simulink model "DRLHevIps"  (R2025b)
settings: Solver=ode23tb  StartTime=0  StopTime=stop_time+1  FixedStep=ts  RelTol=1e-3  AbsTol=1e-4
model workspace (MAT data in the model file):
  BattChrgMax = Simulink.Parameter
  BattChrgMax.Value = -28000
  BattChrgMax.Complexity = 'real'
  BattChrgMax.Dimensions = [1 1]
  BattChrgMax.DataType = 'double'
  BattDischrgMax = Simulink.Parameter
  BattDischrgMax.Value = 28000
  BattDischrgMax.Complexity = 'real'
  BattDischrgMax.Dimensions = [1 1]
  BattDischrgMax.DataType = 'double'
  BrkPrsMax = Simulink.Parameter
  BrkPrsMax.Value = 5000000
  BrkPrsMax.Complexity = 'real'
  BrkPrsMax.Dimensions = [1 1]
  BrkPrsMax.DataType = 'double'
  DiffRatio = Simulink.Parameter
  DiffRatio.Value = 3.267
  DiffRatio.Complexity = 'real'
  DiffRatio.Dimensions = [1 1]
  DiffRatio.DataType = 'double'
  EVSpdLmt = Simulink.Parameter
  EVSpdLmt.Value = 16
  EVSpdLmt.Complexity = 'real'
  EVSpdLmt.Dimensions = [1 1]
  EVSpdLmt.DataType = 'double'
  EngIdle = Simulink.Parameter
  EngIdle.Value = 78.5398163397
  EngIdle.Complexity = 'real'
  EngIdle.Dimensions = [1 1]
  EngIdle.DataType = 'double'
  EngPwr = Simulink.Parameter
  EngPwr.Value = [8377.58040957 15052.6315789 19736.8421053 24421.0526316 29105.2631579 33789.4736842 38473.6842105 43157.8947368 47842.1052632 52526.3157895 57210.5263158 61894.7368421 66578.9473684 71263.1578947 75947.3684211 80631.5789474 85315.7894737 90000]
  EngPwr.Complexity = 'real'
  EngPwr.Dimensions = [1 18]
  EngPwr.DataType = 'double'
  EngSpd = Simulink.Parameter
  EngSpd.Value = [1000 1448.84862461 1712.99052669 1980.33600187 2249.1155588 2517.55970613 2783.89895252 3046.3638066 3303.18477703 3552.59237246 3792.81710154 4022.08947291 4238.63999523 4440.69917715 4626.49752731 4794.26555436 4942.23376695 5068.63267374]
  EngSpd.Complexity = 'real'
  EngSpd.Dimensions = [1 18]
  EngSpd.DataType = 'double'
  EngTrq = Simulink.Parameter
  EngTrq.Value = [80 99.2112225513 110.02568665 117.759751017 123.57514891 128.166058939 131.971967205 135.285068696 138.308475993 141.18967656 144.040766791 146.951280713 149.9967243 153.244568751 156.75874496 160.603298419 164.845657961 169.559869104]
  EngTrq.Complexity = 'real'
  EngTrq.Dimensions = [1 18]
  EngTrq.DataType = 'double'
  EngTrqWhl = Simulink.Parameter
  EngTrqWhl.Value = [87.7908306305 126.105850222 164.420869813 193.843356507 202.735889404 240.750809081 272.197383842 292.721746259 307.117840187 318.924150962 329.429038197 339.950469104 351.800120347 366.619114839 388.284464425 404.750071694]
  EngTrqWhl.Complexity = 'real'
  EngTrqWhl.Dimensions = [1 16]
  EngTrqWhl.DataType = 'double'
  GenMapEff = Simulink.Parameter
  GenMapEff.Value = [60  60  60  60  60  65  60  60  60  60  60  60  60  60  60; 60  78  85  87  88  89  91  91  93  92  92  93  91  90  85; 60  82  88  90  90.5  92.5  94.5  95  95  94.5  93.5  93  93  93  93; 60  82  89  91  91.5  93.5  95  95  94.5  94  93  93  93  93  93; 60  82  88  91  92  94  95  94  94  93  93  93  93  93  93; 60  80  88  90.5  91.5  94  94.5  94  93  93  93  93  93  93  93; 60  78  87  90  90.5  93  94  93  93  93  93  93  93  93  93; 60  75  86  89  90  92  92  92  92  92  92  92  92  92  92; 60  74  84  87.5  89  91  91  91  91  91  91  91  91  91  91; 60  70  81  86  88  88  88  88  88  88  88  88  88  88  88; 60  66  79  86  88  88  88  88  88  88  88  88  88  88  88; 60  66  79  86  88  88  88  88  88  88  88  88  88  88  88]
  GenMapEff.Complexity = 'real'
  GenMapEff.Dimensions = [12 15]
  GenMapEff.DataType = 'double'
  GenMapSpdIndex = Simulink.Parameter
  GenMapSpdIndex.Value = [0 1000 2000 2767.91 3000 4000 5000 6000 7000 8000 9000 10000 11000 12000 13000]
  GenMapSpdIndex.Complexity = 'real'
  GenMapSpdIndex.Dimensions = [1 15]
  GenMapSpdIndex.DataType = 'double'
  GenMapTrqIndex = Simulink.Parameter
  GenMapTrqIndex.Value = [0 14 28 42 56 70 84 98 112 126 140 144.9]
  GenMapTrqIndex.Complexity = 'real'
  GenMapTrqIndex.Dimensions = [1 12]
  GenMapTrqIndex.DataType = 'double'
  GenPwrMax = Simulink.Parameter
  GenPwrMax.Value = 42000
  GenPwrMax.Complexity = 'real'
  GenPwrMax.Dimensions = [1 1]
  GenPwrMax.DataType = 'double'
  GenSpd = Simulink.Parameter
  GenSpd.Value = [0 1000 2000 2767.91 3000 4000 5000 6000 7000 8000 9000 10000 11000 12000 13000 13500]
  GenSpd.Complexity = 'real'
  GenSpd.Dimensions = [1 16]
  GenSpd.DataType = 'double'
  GenTrq = Simulink.Parameter
  GenTrq.Value = [144.9 144.9 144.9 144.9 133.69015219 100.26761416 80.2140913 66.845076102 57.295779513 50.133807073 44.563384068 40.107045657 36.460950596 33.422538051 30.851573585 29.708922712]
  GenTrq.Complexity = 'real'
  GenTrq.Dimensions = [1 16]
  GenTrq.DataType = 'double'
  GenTrqMax = Simulink.Parameter
  GenTrqMax.Value = 144.9
  GenTrqMax.Complexity = 'real'
  GenTrqMax.Dimensions = [1 1]
  GenTrqMax.DataType = 'double'
  MotMapEff = Simulink.Parameter
  MotMapEff.Value = [60  60  60  60  60  65  60  60  60  60  60  60  60  60  60; 60  78  85  87  88  89  91  91  93  92  92  93  91  90  85; 60  82  88  90  90.5  92.5  94.5  95  95  94.5  93.5  93  93  93  93; 60  82  89  91  91.5  93.5  95  95  94.5  94  93  93  93  93  93; 60  82  88  91  92  94  95  94  94  93  93  93  93  93  93; 60  80  88  90.5  91.5  94  94.5  94  93  93  93  93  93  93  93; 60  78  87  90  90.5  93  94  93  93  93  93  93  93  93  93; 60  75  86  89  90  92  92  92  92  92  92  92  92  92  92; 60  74  84  87.5  89  91  91  91  91  91  91  91  91  91  91; 60  70  81  86  88  88  88  88  88  88  88  88  88  88  88; 60  66  79  86  88  88  88  88  88  88  88  88  88  88  88; 60  66  79  86  88  88  88  88  88  88  88  88  88  88  88]
  MotMapEff.Complexity = 'real'
  MotMapEff.Dimensions = [12 15]
  MotMapEff.DataType = 'double'
  MotMapSpdIndex = Simulink.Parameter
  MotMapSpdIndex.Value = [0 1000 2000 2767.91 3000 4000 5000 6000 7000 8000 9000 10000 11000 12000 13000]
  MotMapSpdIndex.Complexity = 'real'
  MotMapSpdIndex.Dimensions = [1 15]
  MotMapSpdIndex.DataType = 'double'
  MotMapTrqIndex = Simulink.Parameter
  MotMapTrqIndex.Value = [0 20 40 60 80 100 120 140 160 180 200 207]
  MotMapTrqIndex.Complexity = 'real'
  MotMapTrqIndex.Dimensions = [1 12]
  MotMapTrqIndex.DataType = 'double'
  MotPwr = Simulink.Parameter
  MotPwr.Value = [0 21676.9893098 43353.9786195 59999.9554804 59999.9999968 60000.0000072 59999.9999863 60000.0000031 59999.9999999 59999.9999989 60000.0000031 59999.9999968 59999.9999947 60000.0000031 60000.000002 60000.0000031]
  MotPwr.Complexity = 'real'
  MotPwr.Dimensions = [1 16]
  MotPwr.DataType = 'double'
  MotSpd = Simulink.Parameter
  MotSpd.Value = [0 1000 2000 2767.91 3000 4000 5000 6000 7000 8000 9000 10000 11000 12000 13000 13500]
  MotSpd.Complexity = 'real'
  MotSpd.Dimensions = [1 16]
  MotSpd.DataType = 'double'
  MotTrq = Simulink.Parameter
  MotTrq.Value = [207 207 207 207 190.9859317 143.2394488 114.591559 95.49296586 81.85111359 71.61972439 63.66197724 57.29577951 52.08707228 47.74648293 44.07367655 42.44131816]
  MotTrq.Complexity = 'real'
  MotTrq.Dimensions = [1 16]
  MotTrq.DataType = 'double'
  Ndiff = Simulink.Parameter
  Ndiff.Value = 3.26774691358
  Ndiff.Complexity = 'real'
  Ndiff.Dimensions = [1 1]
  Ndiff.DataType = 'double'
  Nr1 = Simulink.Parameter
  Nr1.Value = 78
  Nr1.Complexity = 'real'
  Nr1.Dimensions = [1 1]
  Nr1.DataType = 'double'
  Nr2 = Simulink.Parameter
  Nr2.Value = 58
  Nr2.Complexity = 'real'
  Nr2.Dimensions = [1 1]
  Nr2.DataType = 'double'
  Ns1 = Simulink.Parameter
  Ns1.Value = 30
  Ns1.Complexity = 'real'
  Ns1.Dimensions = [1 1]
  Ns1.DataType = 'double'
  Ns2 = Simulink.Parameter
  Ns2.Value = 22
  Ns2.Complexity = 'real'
  Ns2.Dimensions = [1 1]
  Ns2.DataType = 'double'
  NsysWhl = Simulink.Parameter
  NsysWhl.Value = [0 116.077026422 232.154052844 321.290762203 348.231079266 464.308105687 580.385132109 696.462158531 812.539184953 928.616211375 1044.6932378 1160.77026422 1276.84729064 1392.92431706 1509.00134348 1567.0398567]
  NsysWhl.Complexity = 'real'
  NsysWhl.Dimensions = [1 16]
  NsysWhl.DataType = 'double'
  SOCChrgFactor = Simulink.Parameter
  SOCChrgFactor.Value = [84000 8400]
  SOCChrgFactor.Complexity = 'real'
  SOCChrgFactor.Dimensions = [1 2]
  SOCChrgFactor.DataType = 'double'
  SOCerr = Simulink.Parameter
  SOCerr.Value = 20
  SOCerr.Complexity = 'real'
  SOCerr.Dimensions = [1 1]
  SOCerr.DataType = 'double'
  SOCmax = Simulink.Parameter
  SOCmax.Value = 80
  SOCmax.Complexity = 'real'
  SOCmax.Dimensions = [1 1]
  SOCmax.DataType = 'double'
  SOCmin = Simulink.Parameter
  SOCmin.Value = 40
  SOCmin.Complexity = 'real'
  SOCmin.Dimensions = [1 1]
  SOCmin.DataType = 'double'
  SOCtarget = Simulink.Parameter
  SOCtarget.Value = 60
  SOCtarget.Complexity = 'real'
  SOCtarget.Dimensions = [1 1]
  SOCtarget.DataType = 'double'
  SysTrqWhl = Simulink.Parameter
  SysTrqWhl.Value = [1783.29861111 1783.29861111 1783.29861111 1783.29861111 1783.29861111 1474.75423952 1259.40012785 1115.39069983 1012.2626575 935.925866097 877.875007244 833.551841194 800.528640413 777.953591624 767.977827605 770.380717725]
  SysTrqWhl.Complexity = 'real'
  SysTrqWhl.Dimensions = [1 16]
  SysTrqWhl.DataType = 'double'
  k = Simulink.Parameter
  k.Value = 2.6
  k.Complexity = 'real'
  k.Dimensions = [1 1]
  k.DataType = 'double'
values from neighbouring files (symbols this model uses):
  cyc_time = WLTC(:,1)    [mdlrun_time_DG.m]
  cyc_vel = WLTC(:,2)    [mdlrun_time_DG.m]
  en_actsmo = 1    [mdlrun_time_DG.m]
  en_elec = 1    [mdlrun_time_DG.m]
  en_gas = 1    [mdlrun_time_DG.m]
  en_SOCpen = 1    [mdlrun_time_DG.m]
  k_actsmo = 5e-2    (= 0.05)    [mdlrun_time_DG.m]
  k_elec = 1    [mdlrun_time_DG.m]
  k_gas = 1    [mdlrun_time_DG.m]
  k_SOCpen = 1.2    [mdlrun_time_DG.m]
  obs_max = 1e4*[0.0020, 0.0090, 0.0100, 0.0100, 8.4000, 0.0100,                0.0056, 0.1011, 2.8000,      0, 0.0001, 0.0132,                0.0740, 2.6065, 0.0339, 0.0949, 0.0117, 2.4444]    [mdlrun_time_DG.m]
  obs_min = 1e4*[0.0010, 0.0070,      0,      0, 0.8400,      0,                     0, -0.0005,     0, -2.8000,     0, -0.0032               -0.0694, -2.7092, -0.0030,    0, -0.0001, -2.7647]    [mdlrun_time_DG.m]
  Price_elec = 1    [mdlrun_time_DG.m]
  Price_gas = 7.14    [mdlrun_time_DG.m]
  rho_gas = 0.739    [mdlrun_time_DG.m]
  stop_time = cyc_time(end)    [mdlrun_time_DG.m]
  ts = 1    [mdlrun_time_DG.m]
undefined symbols (not defined in the file or in its folder): n_ool, T_ool
libraries: simulink x29, autolibutils x6, slpidlib x2, rllib x2, SignalEditorBlockLib x1, autolibshared x1, autolibhevctrlrcommon x1
(part 1 of 4)
settings Model: DataDictionary=HevIps.sldd  ModifiedByFormat=The MathWorks, Inc.  PauseTimes=23.46  Creator=The MathWorks, Inc.  LastModifiedBy=The MathWorks, Inc.
settings SolverCC: ExtrapolationOrder=1.0  NumberNewtonIterations=20.0  SolverJacobianMethodControl=FullPerturbation  ZeroCrossControl=EnableAll  ZeroCrossAlgorithm=Adaptive  AlgebraicLoopSolver=TrustRegion  AutoInsertRateTranBlk=on  DecoupledContinuousIntegration=on  MinimalZcImpactIntegration=on  MaxZcPerStep=1.0
settings DataIOCC: SaveOutput=off  DSMLogging=off  SaveTime=off  ReturnWorkspaceOutputs=off
settings OptimizationCC: ReuseModelBlockBuffer=off  EfficientMapNaN2IntZero=off
settings DebuggingCC: UnderspecifiedInitializationDetection=Classic  MergeDetectMultiDrivingBlocksExec=none  MaskedZcDiagnostic=none  IgnoredZcDiagnostic=none  UnconnectedInputMsg=warning  UnconnectedOutputMsg=warning  UnconnectedLineMsg=warning  PregeneratedLibrarySubsystemCodeDiagnostic=none  ArithmeticOperatorsInVariantConditions=warning
settings HardwareCC: TargetBitPerPointer=64.0  TargetBitPerSizeT=64.0  TargetBitPerPtrDiffT=64.0  TargetLongLongMode=on  TargetIntDivRoundTo=Zero  TargetEndianess=LittleEndian  TargetWordSize=64.0  TargetHWDeviceType=MATLAB Host  ProdEqTarget=off
settings ModelReferenceCC: UpdateModelReferenceTargets=IfOutOfDate  EnableRefExpFcnMdlSchedulingChecks=on  ModelReferenceMinAlgLoopOccurrences=on  PropagateSignalLabelsOutOfModel=off
settings SFSimCC: SimUseLocalCustomCode=off
settings RTWCC: RTWUseLocalCustomCode=off  GPUComputeCapability=3.5  DLArmComputeVersion=19.05
settings CodeAppCC: MaxIdLength=128.0
settings GRTTargetCC: TargetLangStandard=C89/C90 (ANSI)  CombineOutputUpdateFcns=off  GRTInterface=on
settings ConfigComp: CovMetricSettings=dsw  CovSaveCumulativeToWorkspaceVar=on  CovSaveSingleToWorkspaceVar=on  CovExternalEMLEnable=off

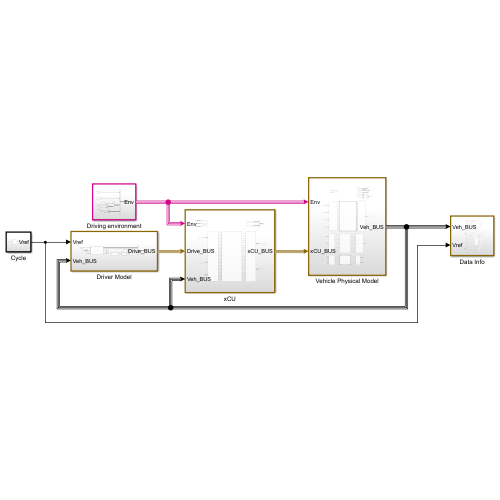
[thumbnail: Simulink's stored preview of the top-level diagram]
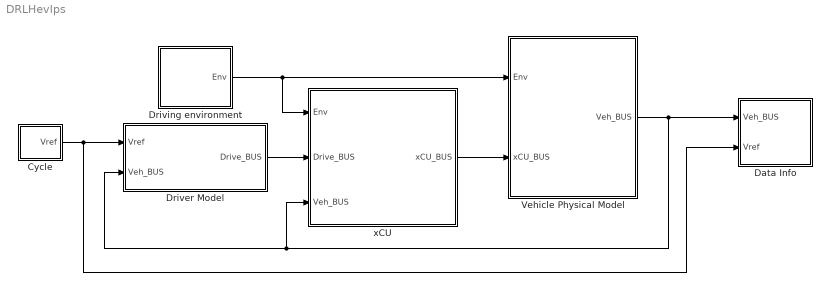
== system DRLHevIps ==
  Cycle : Subsystem
  Data Info : Subsystem
  Driver Model : Subsystem
  Driving environment : Subsystem
  Vehicle Physical Model : Subsystem
  xCU : Subsystem
  wires:
  Driver Model/1(Drive_BUS) -> xCU/2(Drive_BUS)
  Driving environment/1(Env) -> xCU/1(Env), Vehicle Physical Model/1(Env)
  xCU/1(xCU_BUS) -> Vehicle Physical Model/2(xCU_BUS)
  Vehicle Physical Model/1(Veh_BUS) -> Data Info/1(Veh_BUS), Driver Model/2(Veh_BUS), xCU/3(Veh_BUS)
  Cycle/1(Vref) -> Data Info/2(Vref), Driver Model/1(Vref)

== system DRLHevIps/Cycle ==
  1-D Lookup Table : Lookup_n-D  NumberOfTableDimensions=1  BreakpointsForDimension1=cyc_time  Table=cyc_vel  ExtrapMethod=Clip  UseLastTableValue=on  InternalRulePriority=Speed  RndMeth=Simplest
  Clock : Clock
  Gain : Gain  Gain=1/3.6
  Vref : Outport
  wires:
  1-D Lookup Table/1 -> Gain/1
  Clock/1 -> 1-D Lookup Table/1
  Gain/1 -> Vref/1

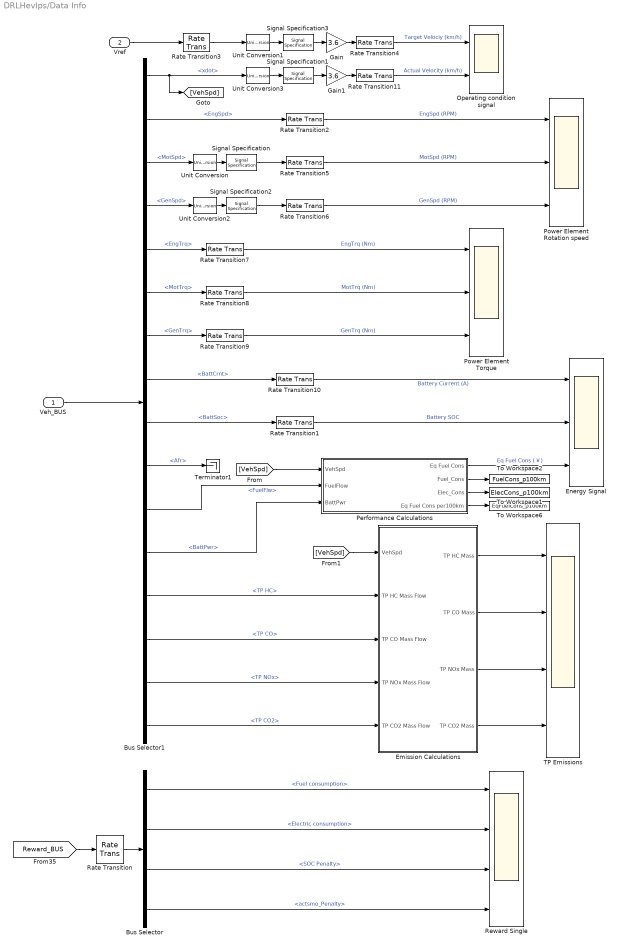
== system DRLHevIps/Data Info ==
  Veh_BUS : Inport
  Vref : Inport  Port=2
  Bus Selector : BusSelector  OutputSignals=Reward Single.Fuel consumption,Reward Single.Electric consumption,Reward Single.SOC Penalty,Reward Single.actsmo_Penalty
  Bus Selector1 : BusSelector  OutputSignals=Veh.xdot,Eng.EngFdbkOut.EngSpd,Veh.MotSpd,Veh.GenSpd,Eng.EngFdbkOut.EngTrq,Elec.MotTrq,Elec.GenTrq,Elec.BattCrnt,Elec.BattSoc,Eng.EngFdbkOut.Afr,Eng.EngFdbkOut.FuelFlw,Elec.BattPwr,Eng.EngFdbkOut.TP HC,Eng.EngFdbkOut.TP CO,Eng.EngFdbkOut.TP NOx,Eng.EngFdbkOut.TP CO2
  Emission Calculations : Subsystem
  Energy Signal : Scope  NumInputPorts=3
      settings: ActiveDisplayYMinimum=-177.98676383868633  ActiveDisplayYMaximum=172.65436797964097  DataLoggingVariableName=ScopeData4
  Gain : Gain  Gain=3.6
  Gain1 : Gain  Gain=3.6
  Operating condition signal : Scope  NumInputPorts=2
      settings: SampleTime=0.1  ActiveDisplayYMinimum=-16.412529630927349  ActiveDisplayYMaximum=147.71250329232529
  Performance Calculations : Subsystem
  Power Element Rotation speed : Scope  NumInputPorts=3
      settings: ActiveDisplayYMinimum=-427.89722446119362  ActiveDisplayYMaximum=3645.4520462760661  DataLoggingVariableName=ScopeData6
  Power Element Torque : Scope  NumInputPorts=3
      settings: ActiveDisplayYMinimum=-52.991599192001743  ActiveDisplayYMaximum=152.76942101093081  DataLoggingVariableName=ScopeData3
  Rate Transition : RateTransition
  Rate Transition{1..11} (11 alike) : RateTransition  Deterministic=off
  Reward Single : Scope  NumInputPorts=4
      settings: ActiveDisplayYMinimum=-0.003792108734088237  ActiveDisplayYMaximum=0.034128819098233433  DataLoggingVariableName=ScopeData2
  Signal Specification : SignalSpecification  Unit=rpm
  Signal Specification1 : SignalSpecification  Unit=m/s
  Signal Specification2 : SignalSpecification  Unit=rpm
  Signal Specification3 : SignalSpecification  Unit=m/s
  TP Emissions : Scope  NumInputPorts=4
      settings: SampleTime=0.1  ActiveDisplayYMinimum=-5.5836894521367283E-5  ActiveDisplayYMaximum=0.00050253205069230569
  Terminator1 : Terminator
  To Workspace1 : ToWorkspace  VariableName=ElecCons_p100km  SampleTime=-1
  To Workspace2 : ToWorkspace  VariableName=FuelCons_p100km  SampleTime=-1
  To Workspace6 : ToWorkspace  VariableName=EqFuelCons_p100km  SampleTime=-1
  Unit Conversion{,1..3} (4 alike) : UnitConversion
  wires:
  Bus Selector1/7 -> Rate Transition9/1  "<GenTrq>"
  Rate Transition6/1 -> Power Element Rotation speed/3  "GenSpd (RPM)"
  Rate Transition9/1 -> Power Element Torque/3  "GenTrq (Nm)"
  Rate Transition8/1 -> Power Element Torque/2  "MotTrq (Nm)"
  Rate Transition5/1 -> Power Element Rotation speed/2  "MotSpd (RPM)"
  Bus Selector1/12 -> Performance Calculations/3(BattPwr)  "<BattPwr>"
  Bus Selector1/13 -> Emission Calculations/2(TP HC Mass Flow)  "<TP HC>"
  Bus Selector1/6 -> Rate Transition8/1  "<MotTrq>"
  Rate Transition3/1 -> Unit Conversion1/1
  Rate Transition1/1 -> Energy Signal/2  "Battery SOC"
  Unit Conversion/1 -> Signal Specification/1
  Performance Calculations/2(Fuel_Cons) -> To Workspace2/1
  Bus Selector1/2 -> Rate Transition2/1  "<EngSpd>"
  Rate Transition2/1 -> Power Element Rotation speed/1  "EngSpd (RPM)"
  Bus Selector1/15 -> Emission Calculations/4(TP NOx Mass Flow)  "<TP NOx>"
  Unit Conversion1/1 -> Signal Specification3/1
  Performance Calculations/1(Eq Fuel Cons) -> Energy Signal/3  "Eq Fuel Cons (￥)"
  Signal Specification2/1 -> Rate Transition6/1
  Rate Transition10/1 -> Energy Signal/1  "Battery Current (A)"
  [VehSpd] -> Performance Calculations/1(VehSpd)
  Emission Calculations/4(TP CO2 Mass) -> TP Emissions/4
  Rate Transition7/1 -> Power Element Torque/1  "EngTrq (Nm)"
  Bus Selector1/10 -> Terminator1/1  "<Afr>"
  Bus Selector1/3 -> Unit Conversion/1  "<MotSpd>"
  Bus Selector1/4 -> Unit Conversion2/1  "<GenSpd>"
  Bus Selector1/16 -> Emission Calculations/5(TP CO2 Mass Flow)  "<TP CO2>"
  Bus Selector1/8 -> Rate Transition10/1  "<BattCrnt>"
  Bus Selector1/9 -> Rate Transition1/1  "<BattSoc>"
  Veh_BUS/1 -> Bus Selector1/1
  Rate Transition4/1 -> Operating condition signal/1  "Target Velociy (km/h)"
  Bus Selector1/1 -> Unit Conversion3/1, [VehSpd]  "<xdot>"
  Signal Specification/1 -> Rate Transition5/1
  Bus Selector1/11 -> Performance Calculations/2(FuelFlow)  "<FuelFlw>"
  Vref/1 -> Rate Transition3/1
  [VehSpd] -> Emission Calculations/1(VehSpd)
  Emission Calculations/2(TP CO Mass) -> TP Emissions/2
  Bus Selector1/5 -> Rate Transition7/1  "<EngTrq>"
  Emission Calculations/1(TP HC Mass) -> TP Emissions/1
  Bus Selector1/14 -> Emission Calculations/3(TP CO Mass Flow)  "<TP CO>"
  Emission Calculations/3(TP NOx Mass) -> TP Emissions/3
  Unit Conversion2/1 -> Signal Specification2/1
  Gain/1 -> Rate Transition4/1
  Signal Specification3/1 -> Gain/1
  Signal Specification1/1 -> Gain1/1
  Gain1/1 -> Rate Transition11/1
  Unit Conversion3/1 -> Signal Specification1/1
  Rate Transition11/1 -> Operating condition signal/2  "Actual Velocity (km/h)"
  [Reward_BUS] -> Rate Transition/1
  Bus Selector/1 -> Reward Single/1  "<Fuel consumption>"
  Rate Transition/1 -> Bus Selector/1
  Bus Selector/2 -> Reward Single/2  "<Electric consumption>"
  Bus Selector/3 -> Reward Single/3  "<SOC Penalty>"
  Bus Selector/4 -> Reward Single/4  "<actsmo_Penalty>"
  Performance Calculations/3(Elec_Cons) -> To Workspace1/1
  Performance Calculations/4(Eq Fuel Cons per100km) -> To Workspace6/1

== system DRLHevIps/Driver Model ==
  Vref : Inport
  Veh_BUS : Inport  Port=2
  Bus Creator1 : BusCreator  Inputs=2
  Bus Selector : BusSelector  OutputSignals=Veh.xdot
  Constant : Constant  Value=false
  Data Type Conversion : DataTypeConversion  OutDataTypeStr=boolean  SaturateOnIntegerOverflow=off  RndMeth=Floor
  Ground : Ground
  Ignition Switch Profile : SignalEditorBlockLib/Signal Editor  FileName=IginitionSwitchProfile.mat  ActiveScenario=Group_1  ActiveSignal=IGSW  IsBus=off  OutputBusObjectStr=Bus: BusObject  SampleTime=0  OutputAfterFinalValue=Extrapolation  Unit=inherit  PreserveSignalName=on  ApplySigPropsToAllScenarios=on  ApplySigPropsToAllSignals=off  SignalPropertySource=Dialog parameters
  Longitudinal Driver Model : autolibshared/Longitudinal Driver  extAccelOvr=off  extDecelOvr=off  extAccelHld=off  extDecelHld=off  extAccelZero=off  extDecelZero=off  cntrlType=Predictive  shftType=Reverse, Neutral, Drive  velUnits=m/s  gearOut=off  Kp=2.5  Ki=2.5  Kff=0  Kg=0  VehVelVec=[0 100]  KffVec=[.1 .1]  KpVec=[10 10]  KiVec=[5 5]  KgVec=[0 0]  m=1500  Kpt=10000  tau=0.12  L=4  aR=160  bR=1  cR=0.36  g=9.81  vnom=5  Kaw=1  tauerr=0  tauPt=2  GearInit=0  tShift=.1  pdlVec=[0.1 0.4 0.5 0.9]  upShftTbl=[-1 12.9375 26.4375 39.9375 51.18749999999999 62.4375 72.84375 83.25;-1 16.3125 29.8125 43.3125 54.5624 65.8125 76.78125 87.75;-1 19.6875 33.1875 46.68749999999999 57.9375 69.1875 80.71875 92.25;-1 33 52.5 77.25 100.5 138.75 161.875 185]  dwnShftTbl=[1 9.5625 23.0625 36.5625 47.8125 59.0625 68.90625 78.75;1 12.9375 26.4375 39.9375 51.18749999999999 62.4375 72.84375 83.25;1 16.3125 29.8125 43.3125 54.562499 65.8125 76.78125 87.75;1 19.6875 33.1875 46.68749999999999 57.9375 69.1875 80.71875 92.25]  tClutch=.5  tRev=.5  tPark=120  aMode=1  UpGearVec="[0  1  2  3  4  5  6  7]"  DownGearVec="[1  2  3  4  5  6  7  8]"
  Manual Switch : ManualSwitch
  Terminator : Terminator
  Terminator1 : Terminator
  Drive_BUS : Outport  VectorParamsAs1DForOutWhenUnconnected=off
  wires:
  Veh_BUS/1 -> Bus Selector/1
  Bus Creator1/1 -> Drive_BUS/1
  Constant/1 -> Manual Switch/1
  Ignition Switch Profile/1 -> Data Type Conversion/1
  Data Type Conversion/1 -> Manual Switch/2
  Manual Switch/1 -> Bus Creator1/2  "IgSw"
  Longitudinal Driver Model/3 -> Terminator1/1  "Dec"
  Ground/1 -> Longitudinal Driver Model/3
  Longitudinal Driver Model/1 -> Bus Creator1/1  "Info"
  Vref/1 -> Longitudinal Driver Model/1  "xdotref"
  Longitudinal Driver Model/2 -> Terminator/1  "Acc"
  Bus Selector/1 -> Longitudinal Driver Model/2  "<xdot>"

== system DRLHevIps/Driving environment ==
  Bus Creator : BusCreator  Inputs=4
  Bus Creator3 : BusCreator  Inputs=3
  Bus Creator4 : BusCreator  Inputs=2
  Bus Creator5 : BusCreator  Inputs=2
  Constant2 : Constant  Value=0
  Constant3 : Constant  Value=0
  Constant6 : Constant  Value=300
  Constant7 : Constant  Value=101325
  Ground{,1..3} (4 alike) : Ground
  Env : Outport  VectorParamsAs1DForOutWhenUnconnected=off
  wires:
  Ground1/1 -> Bus Creator3/3  "wind_z"
  Bus Creator3/1 -> Bus Creator/4  "Wind"
  Ground2/1 -> Bus Creator5/1  "lam_mu_x"
  Constant2/1 -> Bus Creator4/1  "Grade"
  Constant7/1 -> Bus Creator/2  "Baro"
  Bus Creator4/1 -> Bus Creator/3  "Ground"
  Constant3/1 -> Bus Creator3/1  "wind_x"
  Ground/1 -> Bus Creator3/2  "wind_y"
  Bus Creator5/1 -> Bus Creator4/2  "Ground_mu"
  Bus Creator/1 -> Env/1  "Environment"
  Constant6/1 -> Bus Creator/1  "Temp"
  Ground3/1 -> Bus Creator5/2  "lam_mu_y"

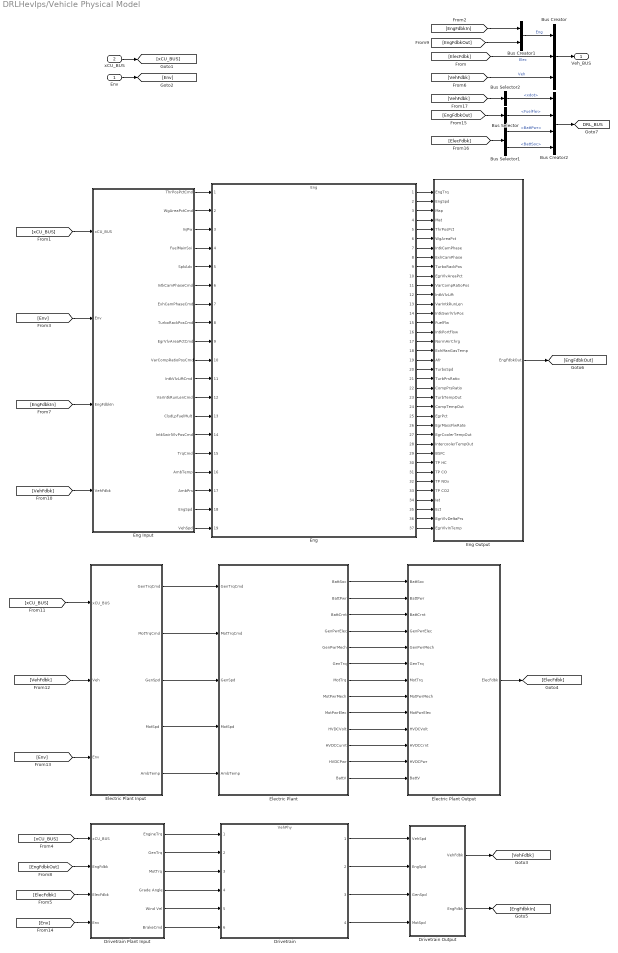
== system DRLHevIps/Vehicle Physical Model ==
  Env : Inport
  xCU_BUS : Inport  Port=2
  Bus Creator : BusCreator  Inputs=3
  Bus Creator1 : BusCreator  Inputs=2
  Bus Creator2 : BusCreator  Inputs=4
  Bus Selector : BusSelector  OutputSignals=FuelFlw
  Bus Selector1 : BusSelector  OutputSignals=BattPwr,BattSoc
  Bus Selector2 : BusSelector  OutputSignals=xdot
  Drivetrain : ModelReference  ModelNameDialog=VehPhy.slx  ModelReferenceVersion=14.29  InputSignalHandling=Zero-order hold
  Drivetrain Output : Subsystem
  Drivetrain Plant Input : Subsystem
  Electric Plant : Subsystem
  Electric Plant Input : Subsystem
  Electric Plant Output : Subsystem
  Eng : ModelReference  ModelNameDialog=Eng.slx  ModelReferenceVersion=13.15
  Eng Input : Subsystem
  Eng Output : Subsystem
  Veh_BUS : Outport  VectorParamsAs1DForOutWhenUnconnected=off
  tag scope: DRL_BUS=global
  wires:
  Eng Input/2(WgAreaPctCmd) -> Eng/2
  Eng/19 -> Eng Output/19(Afr)
  Electric Plant/5(GenPwrMech) -> Electric Plant Output/5(GenPwrMech)
  [VehFdbk] -> Bus Creator/3  "Veh"
  Eng/15 -> Eng Output/15(FuelFlw)
  [xCU_BUS] -> Drivetrain Plant Input/1(xCU_BUS)
  Electric Plant/1(BattSoc) -> Electric Plant Output/1(BattSoc)
  Electric Plant Input/1(GenTrqCmd) -> Electric Plant/1(GenTrqCmd)
  Electric Plant Input/4(MotSpd) -> Electric Plant/4(MotSpd)
  [EngFdbkIn] -> Eng Input/3(EngFdbkIn)
  Drivetrain Plant Input/3(MotTrq) -> Drivetrain/3
  [Env] -> Electric Plant Input/3(Env)
  [xCU_BUS] -> Electric Plant Input/1(xCU_BUS)
  Electric Plant Output/1(ElecFdbk) -> [ElecFdbk]
  Eng Input/18(EngSpd) -> Eng/18
  Eng/2 -> Eng Output/2(EngSpd)
  Drivetrain Plant Input/2(GenTrq) -> Drivetrain/2
  Eng/22 -> Eng Output/22(CompPrsRatio)
  Drivetrain Plant Input/4(Grade Angle) -> Drivetrain/4
  Eng/31 -> Eng Output/31(TP CO)
  Eng/17 -> Eng Output/17(NormAirChrg)
  Eng/35 -> Eng Output/35(Ect)
  Eng/7 -> Eng Output/7(IntkCamPhase)
  Eng/21 -> Eng Output/21(TurbPrsRatio)
  Electric Plant/4(GenPwrElec) -> Electric Plant Output/4(GenPwrElec)
  Eng/14 -> Eng Output/14(IntkSwirlVlvPos)
  Eng/28 -> Eng Output/28(IntercoolerTempOut)
  Eng/9 -> Eng Output/9(TurboRackPos)
  Electric Plant/8(MotPwrMech) -> Electric Plant Output/8(MotPwrMech)
  Electric Plant/2(BattPwr) -> Electric Plant Output/2(BattPwr)
  Eng Input/19(VehSpd) -> Eng/19
  [EngFdbkIn] -> Bus Creator1/1
  Eng Input/6(IntkCamPhaseCmd) -> Eng/6
  Eng/24 -> Eng Output/24(CompTempOut)
  Bus Creator/1 -> Veh_BUS/1
  Eng/20 -> Eng Output/20(TurboSpd)
  Drivetrain Output/2(EngFdbk) -> [EngFdbkIn]
  Electric Plant/12(HVDCPwr) -> Electric Plant Output/12(HVDCPwr)
  xCU_BUS/1 -> [xCU_BUS]
  Eng/37 -> Eng Output/37(EgrVlvInTemp)
  Eng/6 -> Eng Output/6(WgAreaPct)
  Eng Input/9(EgrVlvAreaPctCmd) -> Eng/9
  Eng Input/11(IntkVlvLiftCmd) -> Eng/11
  Eng Input/5(SpkAdv) -> Eng/5
  Drivetrain Plant Input/5(Wind Vel) -> Drivetrain/5
  Electric Plant/3(BattCrnt) -> Electric Plant Output/3(BattCrnt)
  Drivetrain/3 -> Drivetrain Output/3(GenSpd)
  Eng/1 -> Eng Output/1(EngTrq)
  Eng/30 -> Eng Output/30(TP HC)
  Eng/13 -> Eng Output/13(VarIntkRunLen)
  [VehFdbk] -> Eng Input/4(VehFdbk)
  Eng/10 -> Eng Output/10(EgrVlvAreaPct)
  Eng Output/1(EngFdbkOut) -> [EngFdbkOut]
  Eng Input/12(VarIntkRunLenCmd) -> Eng/12
  [Env] -> Drivetrain Plant Input/4(Env)
  Eng Input/13(ClsdLpFuelMult) -> Eng/13
  Eng/16 -> Eng Output/16(IntkPortFlow)
  Drivetrain/2 -> Drivetrain Output/2("EngSpd ")
  Drivetrain Plant Input/6(BrakeCmd) -> Drivetrain/6
  Eng/32 -> Eng Output/32(TP NOx)
  Drivetrain Output/1(VehFdbk) -> [VehFdbk]
  Eng/33 -> Eng Output/33(TP CO2)
  Drivetrain Plant Input/1(EngineTrq) -> Drivetrain/1
  Eng/18 -> Eng Output/18(ExhManGasTemp)
  Eng Input/16(AmbTemp) -> Eng/16
  Eng/11 -> Eng Output/11(VarCompRatioPos)
  Electric Plant/9(MotPwrElec) -> Electric Plant Output/9(MotPwrElec)
  Eng Input/3(InjPw) -> Eng/3
  [xCU_BUS] -> Eng Input/1(xCU_BUS)
  [ElecFdbk] -> Drivetrain Plant Input/3(ElecFdbk)
  Eng Input/17(AmbPrs) -> Eng/17
  Env/1 -> [Env]
  Drivetrain/4 -> Drivetrain Output/4(MotSpd)
  Electric Plant Input/2(MotTrqCmd) -> Electric Plant/2(MotTrqCmd)
  Eng/8 -> Eng Output/8(ExhCamPhase)
  Eng Input/1(ThrPosPctCmd) -> Eng/1
  Electric Plant Input/5(AmbTemp) -> Electric Plant/5(AmbTemp)
  Eng Input/15(TrqCmd) -> Eng/15
  Eng/26 -> Eng Output/26(EgrMassFlwRate)
  Eng Input/7(ExhCamPhaseCmd) -> Eng/7
  Eng/36 -> Eng Output/36(EgrVlvDeltaPrs)
  Eng/23 -> Eng Output/23(TurbTempOut)
  Eng/34 -> Eng Output/34(Iat)
  [VehFdbk] -> Electric Plant Input/2(Veh)
  Eng Input/14(IntkSwirlVlvPosCmd) -> Eng/14
  Eng/5 -> Eng Output/5(ThrPosPct)
  Eng/25 -> Eng Output/25(EgrPct)
  Drivetrain/1 -> Drivetrain Output/1(VehSpd)
  Eng/29 -> Eng Output/29(BSFC)
  Electric Plant/7(MotTrq) -> Electric Plant Output/7(MotTrq)
  [EngFdbkOut] -> Drivetrain Plant Input/2(EngFdbk)
  Electric Plant/13(BattV) -> Electric Plant Output/13(BattV)
  Eng/3 -> Eng Output/3(Map)
  Eng Input/4(FuelMainSoi) -> Eng/4
  Eng/27 -> Eng Output/27(EgrCoolerTempOut)
  [ElecFdbk] -> Bus Creator/2  "Elec"
  Eng Input/10(VarCompRatioPosCmd) -> Eng/10
  Electric Plant Input/3(GenSpd) -> Electric Plant/3(GenSpd)
  Eng/12 -> Eng Output/12(IntkVlvLift)
  [Env] -> Eng Input/2(Env)
  Eng Input/8(TurboRackPosCmd) -> Eng/8
  Eng/4 -> Eng Output/4(Mat)
  Electric Plant/11(HVDCCurnt) -> Electric Plant Output/11(HVDCCrnt)
  Electric Plant/6(GenTrq) -> Electric Plant Output/6(GenTrq)
  Bus Creator1/1 -> Bus Creator/1  "Eng"
  [EngFdbkOut] -> Bus Creator1/2
  Electric Plant/10(HVDCVolt) -> Electric Plant Output/10(HVDCVolt)
  Bus Selector2/1 -> Bus Creator2/1  "<xdot>"
  [EngFdbkOut] -> Bus Selector/1
  Bus Selector1/1 -> Bus Creator2/3  "<BattPwr>"
  Bus Selector/1 -> Bus Creator2/2  "<FuelFlw>"
  [ElecFdbk] -> Bus Selector1/1
  Bus Creator2/1 -> [DRL_BUS]
  [VehFdbk] -> Bus Selector2/1
  Bus Selector1/2 -> Bus Creator2/4  "<BattSoc>"

== system DRLHevIps/xCU ==
  Env : Inport
  Drive_BUS : Inport  Port=2
  Veh_BUS : Inport  Port=3
  Bus Creator : BusCreator  Inputs=2
  xCU : Subsystem
  xCU Input : Subsystem
  xCU Output : Subsystem
  xCU_BUS : Outport  VectorParamsAs1DForOutWhenUnconnected=off
  wires:
  xCU Input/15(IntkSwirlVlvPos) -> xCU/15(IntkSwirlVlvPos)
  [Env] -> xCU Input/2(Env)
  xCU Input/19(DecCmd) -> xCU/19(DecCmd)
  xCU/4(FuelMainSoi) -> xCU Output/4(FuelMainSoi)
  [ECU_BUS] -> Bus Creator/1  "ECU_BUS"
  xCU Input/1(TrqCmd) -> xCU/1(TrqCmd)
  [Drive_BUS] -> xCU Input/4(Drive_BUS)
  xCU Input/29(BattCrnt) -> xCU/29(BattCrnt)
  Bus Creator/1 -> xCU_BUS/1
  xCU Input/22(Ect) -> xCU/22(Ect)
  xCU/10(VarCompRatioPosCmd) -> xCU Output/10(VarCompRatioPosCmd)
  xCU Input/11(VarCompRatioPos) -> xCU/11(VarCompRatioPos)
  xCU Input/24(EgrInTemp) -> xCU/24(EgrVlvInTemp)
  xCU/19(GenTrqCmd) -> xCU Output/19(GenTrqCmd)
  Veh_BUS/1 -> [Veh_BUS]
  xCU/7(ExhCamPhaseCmd) -> xCU Output/7(ExhCamPhaseCmd)
  xCU Input/18(AccCmd) -> xCU/18(AccCmd)
  xCU Input/3(Map) -> xCU/3(Map)
  xCU Input/9(TurboRackPos) -> xCU/9(TurboRackPos)
  xCU Input/25(VehSpdFdbk) -> xCU/25(VehSpdFdbk)
  xCU/17(EstIntkPortFlw) -> xCU Output/17(EstIntkPortFlw)
  xCU/13(ClsdLpFuelMult) -> xCU Output/13(ClsdLpFuelMult)
  xCU Input/16(TurboSpd) -> xCU/16(TurboSpd)
  Drive_BUS/1 -> [Drive_BUS]
  xCU/9(EgrVlvAreaPctCmd) -> xCU Output/9(EgrVlvAreaPctCmd)
  xCU/18(EngTrqCmd) -> xCU Output/18(EngTrqCmd)
  xCU Input/10(EgrVlvAreaPct) -> xCU/10(EgrVlvAreaPct)
  xCU Input/31(GenSpd) -> xCU/31(GenSpd)
  xCU/2(WgAreaPctCmd) -> xCU Output/2(WgAreaPctCmd)
  [VCU_BUS] -> Bus Creator/2  "VCU_BUS"
  xCU/11(IntkVlvLiftCmd) -> xCU Output/11(IntkVlvLiftCmd)
  xCU Input/2(EngSpd) -> xCU/2(EngSpd)
  xCU Input/12(IntkVlvLift) -> xCU/12(IntkVlvLift)
  xCU/6(IntkCamPhaseCmd) -> xCU Output/6(IntkCamPhaseCmd)
  xCU/15(TrqCmdISC) -> xCU Output/15(TrqCmdISC)
  xCU Input/23(EgrDeltaPrs) -> xCU/23(EgrVlvDeltaPrs)
  xCU Input/34(EngTrqOut) -> xCU/34(EngTrqOut)
  xCU Output/1(ECU_BUS) -> [ECU_BUS]
  xCU/8(TurboRackPosCmd) -> xCU Output/8(TurboRackPosCmd)
  xCU Input/5(ThrPosPct) -> xCU/5(ThrPosPct)
  xCU/20(MotTrqCmd) -> xCU Output/20(MotTrqCmd)
  xCU Input/17(AmbPrs) -> xCU/17(AmbPrs)
  xCU Input/13(VarIntkRunLen) -> xCU/13(VarIntkRunLen)
  xCU Input/33(MotPwrElec) -> xCU/33(MotPwrElec)
  [Veh_BUS] -> xCU Input/3(Veh_BUS)
  xCU Output/2(VCU_BUS) -> [VCU_BUS]
  xCU Input/27(BattSoc) -> xCU/27(BattSoc)
  xCU Input/30(MotSpd) -> xCU/30(MotSpd)
  xCU Input/4(Mat) -> xCU/4(Mat)
  xCU/21(BrakeCmd) -> xCU Output/21(BrakeCmd)
  xCU Input/7(IntkCamPhase) -> xCU/7(IntkCamPhase)
  xCU/14(IntkSwirlVlvPosCmd) -> xCU Output/14(IntkSwirlVlvPosCmd)
  xCU Input/26(EngSpdFdbk) -> xCU/26(EngSpdFdbk)
  xCU/1(ThrPosPctCmd) -> xCU Output/1(ThrPosPctCmd)
  xCU Input/8(ExhCamPhase) -> xCU/8(ExhCamPhase)
  xCU Input/20(IgSw) -> xCU/20(IgSw)
  xCU Input/6(WgAreaPct) -> xCU/6(WgAreaPct)
  xCU/12(VarIntkRunLenCmd) -> xCU Output/12(VarIntkRunLenCmd)
  xCU/3(InjPw) -> xCU Output/3(InjPw)
  xCU Input/21(Iat) -> xCU/21(Iat)
  [VCU_BUS] -> xCU Input/1(VCU_BUS)
  xCU Input/28(BattPwr) -> xCU/28(BattPwr)
  xCU/16(LoadCmd) -> xCU Output/16(LoadCmd)
  xCU/5(SpdAdv) -> xCU Output/5(SpkAdv)
  xCU Input/32(GenPwrElec) -> xCU/32(GenPwrElec)
  Env/1 -> [Env]
  xCU Input/14(Afr) -> xCU/14(Afr)

== system DRLHevIps/Data Info/Emission Calculations ==
  VehSpd : Inport
  TP HC Mass Flow : Inport  Port=2
  TP CO Mass Flow : Inport  Port=3
  TP NOx Mass Flow : Inport  Port=4
  TP CO2 Mass Flow : Inport  Port=5
  Integrator{,1..4} (5 alike) : Integrator
  Kg to g : Gain  Gain=1000
  "Kg to g " : Gain  Gain=1000
  "Kg to g  " : Gain  Gain=1000
  "Kg to g   " : Gain  Gain=1000
  L/100 Km Calc{,1..3} (4 alike) : Product  Inputs=/*
  Rate Transition{,1..3} (4 alike) : RateTransition  Deterministic=off
  Saturation1 : Saturate  UpperLimit=Inf  LowerLimit=1
  m to km : Gain  Gain=0.001
  TP HC Mass : Outport  VectorParamsAs1DForOutWhenUnconnected=off
  TP CO Mass : Outport  Port=2  VectorParamsAs1DForOutWhenUnconnected=off
  TP NOx Mass : Outport  Port=3  VectorParamsAs1DForOutWhenUnconnected=off
  TP CO2 Mass : Outport  Port=4  VectorParamsAs1DForOutWhenUnconnected=off
  wires:
  L/100 Km Calc/1 -> Rate Transition/1
  VehSpd/1 -> Integrator/1
  Saturation1/1 -> L/100 Km Calc/1, L/100 Km Calc1/1, L/100 Km Calc2/1, L/100 Km Calc3/1
  TP HC Mass Flow/1 -> Integrator1/1
  Integrator1/1 -> Kg to g/1
  Integrator/1 -> m to km/1
  Kg to g/1 -> L/100 Km Calc/2
  TP CO Mass Flow/1 -> Integrator2/1
  Integrator2/1 -> "Kg to g "/1
  "Kg to g "/1 -> L/100 Km Calc1/2
  TP NOx Mass Flow/1 -> Integrator3/1
  Integrator3/1 -> "Kg to g  "/1
  "Kg to g  "/1 -> L/100 Km Calc2/2
  L/100 Km Calc1/1 -> Rate Transition1/1
  L/100 Km Calc2/1 -> Rate Transition2/1
  TP CO2 Mass Flow/1 -> Integrator4/1
  Integrator4/1 -> "Kg to g   "/1
  "Kg to g   "/1 -> L/100 Km Calc3/2
  L/100 Km Calc3/1 -> Rate Transition3/1
  m to km/1 -> Saturation1/1
  Rate Transition/1 -> TP HC Mass/1  "TP HC Mass (g/km)"
  Rate Transition1/1 -> TP CO Mass/1  "TP CO Mass (g/km)"
  Rate Transition2/1 -> TP NOx Mass/1  "TP NOx Mass (g/km)"
  Rate Transition3/1 -> TP CO2 Mass/1  "TP CO2 Mass (g/km)"

== system DRLHevIps/Data Info/Performance Calculations ==
  VehSpd : Inport
  FuelFlow : Inport  Port=2
  BattPwr : Inport  Port=3
  Abs : Abs  SaturateOnIntegerOverflow=off
  Add : Sum
  Add1 : Sum
  Gain : Gain  Gain=100
  Gain1 : Gain  Gain=100
  Integrator : Integrator
  Integrator1 : Integrator
  Integrator2 : Integrator
  J2kwh : Gain  Gain=1/(3.6e6)
  Price_elec : Gain  Gain=Price_elec
  Price_gas : Gain  Gain=Price_gas
  Product : Product  Inputs=*/
  Product1 : Product  Inputs=*/
  Rate Transition{1..4} (4 alike) : RateTransition  Deterministic=off
  Saturation : Saturate  UpperLimit=Inf  LowerLimit=1
  Saturation1 : Saturate  UpperLimit=Inf  LowerLimit=1
  kg2L : Gain  Gain=1/rho_gas
  m2km : Gain  Gain=1/1000
  Eq Fuel Cons : Outport  VectorParamsAs1DForOutWhenUnconnected=off
  Fuel_Cons : Outport  Port=2  VectorParamsAs1DForOutWhenUnconnected=off
  Elec_Cons : Outport  Port=3  VectorParamsAs1DForOutWhenUnconnected=off
  Eq Fuel Cons per100km : Outport  Port=4  VectorParamsAs1DForOutWhenUnconnected=off
  wires:
  Integrator/1 -> m2km/1
  Integrator1/1 -> kg2L/1
  FuelFlow/1 -> Integrator1/1
  BattPwr/1 -> Integrator2/1
  Abs/1 -> Integrator/1
  VehSpd/1 -> Abs/1
  m2km/1 -> [D_km]
  kg2L/1 -> Price_gas/1
  [D_km] -> Saturation/1
  Saturation/1 -> Product/2
  [Fuel_price] -> Product/1
  Product/1 -> Gain/1
  Gain/1 -> Add/1, Rate Transition2/1
  Integrator2/1 -> J2kwh/1
  J2kwh/1 -> Price_elec/1
  Saturation1/1 -> Product1/2
  [D_km] -> Saturation1/1
  [Energy_price] -> Product1/1
  Product1/1 -> Gain1/1
  Gain1/1 -> Add/2, Rate Transition4/1
  Add/1 -> Rate Transition3/1  "Eq_Cons"
  Rate Transition3/1 -> Eq Fuel Cons per100km/1
  [Energy_price] -> Add1/2
  [Fuel_price] -> Add1/1
  Add1/1 -> Rate Transition1/1
  Rate Transition1/1 -> Eq Fuel Cons/1
  Rate Transition2/1 -> Fuel_Cons/1
  Rate Transition4/1 -> Elec_Cons/1
  Price_gas/1 -> [Fuel_price]
  Price_elec/1 -> [Energy_price]

== system DRLHevIps/Vehicle Physical Model/Drivetrain Output ==
  VehSpd : Inport
  "EngSpd " : Inport  Port=2
  GenSpd : Inport  Port=3
  MotSpd : Inport  Port=4
  Bus Creator1 : BusCreator  Inputs=3
  Bus Creator3 : BusCreator  Inputs=1
  VehFdbk : Outport  VectorParamsAs1DForOutWhenUnconnected=off
  EngFdbk : Outport  Port=2  VectorParamsAs1DForOutWhenUnconnected=off
  wires:
  Bus Creator1/1 -> VehFdbk/1  "VehFdbk"
  VehSpd/1 -> Bus Creator1/1
  "EngSpd "/1 -> Bus Creator3/1  "EngSpd"
  Bus Creator3/1 -> EngFdbk/1  "EngFdbk"
  GenSpd/1 -> Bus Creator1/2  "GenSpd"
  MotSpd/1 -> Bus Creator1/3  "MotSpd"

== system DRLHevIps/Vehicle Physical Model/Drivetrain Plant Input ==
  xCU_BUS : Inport
  EngFdbk : Inport  Port=2
  ElecFdbk : Inport  Port=3
  Env : Inport  Port=4
  Bus Selector : BusSelector  OutputSignals=VCU_BUS.BrakeCmd
  Bus Selector1 : BusSelector  OutputSignals=GenTrq,MotTrq
  Bus Selector2 : BusSelector  OutputSignals=EngTrq
  Bus Selector3 : BusSelector  OutputSignals=Ground.Grade,Wind.wind_x
  Engine Flex Plate Dynamics : TransferFcn  Denominator=[0.05 1]
  First Order Hold : FirstOrderHold  ErrorTolerance=inf  AllowContinuousInput=on
  EngineTrq : Outport  VectorParamsAs1DForOutWhenUnconnected=off
  GenTrq : Outport  Port=2  VectorParamsAs1DForOutWhenUnconnected=off
  MotTrq : Outport  Port=3  VectorParamsAs1DForOutWhenUnconnected=off
  Grade Angle : Outport  Port=4  VectorParamsAs1DForOutWhenUnconnected=off
  Wind Vel : Outport  Port=5  VectorParamsAs1DForOutWhenUnconnected=off
  BrakeCmd : Outport  Port=6  VectorParamsAs1DForOutWhenUnconnected=off
  wires:
  xCU_BUS/1 -> Bus Selector/1
  Engine Flex Plate Dynamics/1 -> EngineTrq/1  "EngineTrq"
  Bus Selector2/1 -> Engine Flex Plate Dynamics/1  "<EngTrq>"
  EngFdbk/1 -> Bus Selector2/1
  Bus Selector/1 -> First Order Hold/1  "<BrakeCmd>"
  First Order Hold/1 -> BrakeCmd/1  "BrakeCntrlCmd"
  ElecFdbk/1 -> Bus Selector1/1
  Env/1 -> Bus Selector3/1
  Bus Selector1/1 -> GenTrq/1  "<GenTrq>"
  Bus Selector1/2 -> MotTrq/1  "<MotTrq>"
  Bus Selector3/1 -> Grade Angle/1  "<Grade>"
  Bus Selector3/2 -> Wind Vel/1  "<wind_x>"

== system DRLHevIps/Vehicle Physical Model/Electric Plant ==
  GenTrqCmd : Inport
  MotTrqCmd : Inport  Port=2
  GenSpd : Inport  Port=3
  MotSpd : Inport  Port=4
  AmbTemp : Inport  Port=5
  Bat : ModelReference  ModelNameDialog=Bat.slx  ModelReferenceVersion=16.10
  Battery Discharge Dynamics : TransferFcn  Denominator=[0.01 1]
  Bus Current : Sum
  Gen : ModelReference  ModelNameDialog=Gen.slx  ModelReferenceVersion=14.7
  Generator Coupling Dynamics : TransferFcn  Denominator=[0.0025 1]
  Mot : ModelReference  ModelNameDialog=Mot.slx  ModelReferenceVersion=14.7
  Motor Coupling Dynamics : TransferFcn  Denominator=[0.01 1]
  Product{,1,3..4} (4 alike) : Product
  BattSoc : Outport  VectorParamsAs1DForOutWhenUnconnected=off
  BattPwr : Outport  Port=2  VectorParamsAs1DForOutWhenUnconnected=off
  BattCrnt : Outport  Port=3  VectorParamsAs1DForOutWhenUnconnected=off
  GenPwrElec : Outport  Port=4  VectorParamsAs1DForOutWhenUnconnected=off
  GenPwrMech : Outport  Port=5  VectorParamsAs1DForOutWhenUnconnected=off
  GenTrq : Outport  Port=6  VectorParamsAs1DForOutWhenUnconnected=off
  MotTrq : Outport  Port=7  VectorParamsAs1DForOutWhenUnconnected=off
  MotPwrMech : Outport  Port=8  VectorParamsAs1DForOutWhenUnconnected=off
  MotPwrElec : Outport  Port=9  VectorParamsAs1DForOutWhenUnconnected=off
  HVDCVolt : Outport  Port=10  VectorParamsAs1DForOutWhenUnconnected=off
  HVDCCurnt : Outport  Port=11  VectorParamsAs1DForOutWhenUnconnected=off
  HVDCPwr : Outport  Port=12  VectorParamsAs1DForOutWhenUnconnected=off
  BattV : Outport  Port=13  VectorParamsAs1DForOutWhenUnconnected=off
  wires:
  Product/1 -> GenPwrMech/1  "GenPwrMech"
  Bus Current/1 -> Battery Discharge Dynamics/1, HVDCCurnt/1  "HVDCCrnt"
  Bat/4 -> Gen/3, Product1/2, Mot/3, Product3/2, HVDCVolt/1  "HVDCVolt"
  Product1/1 -> GenPwrElec/1  "GenPwrElec"
  Bat/1 -> BattSoc/1  "BattSoc"
  MotSpd/1 -> Mot/2, Product4/1
  Gen/2 -> Product1/1, Bus Current/1
  MotTrqCmd/1 -> Mot/1
  GenTrqCmd/1 -> Gen/1
  AmbTemp/1 -> Bat/1
  GenSpd/1 -> Gen/2, Product/1
  Mot/1 -> Motor Coupling Dynamics/1
  Gen/1 -> Generator Coupling Dynamics/1
  Generator Coupling Dynamics/1 -> Product/2, GenTrq/1  "GenTrq"
  Mot/2 -> Bus Current/2, Product3/1
  Motor Coupling Dynamics/1 -> Product4/2, MotTrq/1  "MotTrq"
  Product3/1 -> MotPwrElec/1  "MotPwrElec"
  Product4/1 -> MotPwrMech/1  "MotPwrMech"
  Bat/2 -> BattV/1  "BattV"
  Bat/3 -> BattCrnt/1  "BattCrnt"
  Bat/6 -> HVDCPwr/1  "HVDCPwr"
  Bat/5 -> BattPwr/1  "BattPwr"
  Battery Discharge Dynamics/1 -> Bat/2

== system DRLHevIps/Vehicle Physical Model/Electric Plant Input ==
  xCU_BUS : Inport
  Veh : Inport  Port=2
  Env : Inport  Port=3
  Bus Selector : BusSelector  OutputSignals=VCU_BUS.GenTrqCmd,VCU_BUS.MotTrqCmd
  Bus Selector1 : BusSelector  OutputSignals=GenSpd,MotSpd
  Bus Selector2 : BusSelector  OutputSignals=Temp
  First Order Hold : FirstOrderHold  ErrorTolerance=inf  AllowContinuousInput=on
  First Order Hold1 : FirstOrderHold  ErrorTolerance=inf  AllowContinuousInput=on
  GenTrqCmd : Outport  VectorParamsAs1DForOutWhenUnconnected=off
  MotTrqCmd : Outport  Port=2  VectorParamsAs1DForOutWhenUnconnected=off
  GenSpd : Outport  Port=3  VectorParamsAs1DForOutWhenUnconnected=off
  MotSpd : Outport  Port=4  VectorParamsAs1DForOutWhenUnconnected=off
  AmbTemp : Outport  Port=5  VectorParamsAs1DForOutWhenUnconnected=off
  wires:
  First Order Hold1/1 -> MotTrqCmd/1  "MotTrqCmd"
  First Order Hold/1 -> GenTrqCmd/1  "GenTrqCmd"
  xCU_BUS/1 -> Bus Selector/1
  Bus Selector/2 -> First Order Hold1/1  "<MotTrqCmd>"
  Bus Selector/1 -> First Order Hold/1  "<GenTrqCmd>"
  Veh/1 -> Bus Selector1/1
  Env/1 -> Bus Selector2/1
  Bus Selector2/1 -> AmbTemp/1  "<Temp>"
  Bus Selector1/1 -> GenSpd/1  "<GenSpd>"
  Bus Selector1/2 -> MotSpd/1  "<MotSpd>"

== system DRLHevIps/Vehicle Physical Model/Electric Plant Output ==
  BattSoc : Inport
  BattPwr : Inport  Port=2
  BattCrnt : Inport  Port=3
  GenPwrElec : Inport  Port=4
  GenPwrMech : Inport  Port=5
  GenTrq : Inport  Port=6
  MotTrq : Inport  Port=7
  MotPwrMech : Inport  Port=8
  MotPwrElec : Inport  Port=9
  HVDCVolt : Inport  Port=10
  HVDCCrnt : Inport  Port=11
  HVDCPwr : Inport  Port=12
  BattV : Inport  Port=13
  Bus Creator1 : BusCreator  Inputs=13
  ElecFdbk : Outport  VectorParamsAs1DForOutWhenUnconnected=off
  wires:
  Bus Creator1/1 -> ElecFdbk/1  "ElecFdbk"
  BattPwr/1 -> Bus Creator1/2
  BattSoc/1 -> Bus Creator1/1
  BattCrnt/1 -> Bus Creator1/3
  GenTrq/1 -> Bus Creator1/6
  MotTrq/1 -> Bus Creator1/7
  GenPwrElec/1 -> Bus Creator1/4
  GenPwrMech/1 -> Bus Creator1/5
  MotPwrMech/1 -> Bus Creator1/8
  MotPwrElec/1 -> Bus Creator1/9
  HVDCVolt/1 -> Bus Creator1/10
  HVDCCrnt/1 -> Bus Creator1/11
  HVDCPwr/1 -> Bus Creator1/12
  BattV/1 -> Bus Creator1/13

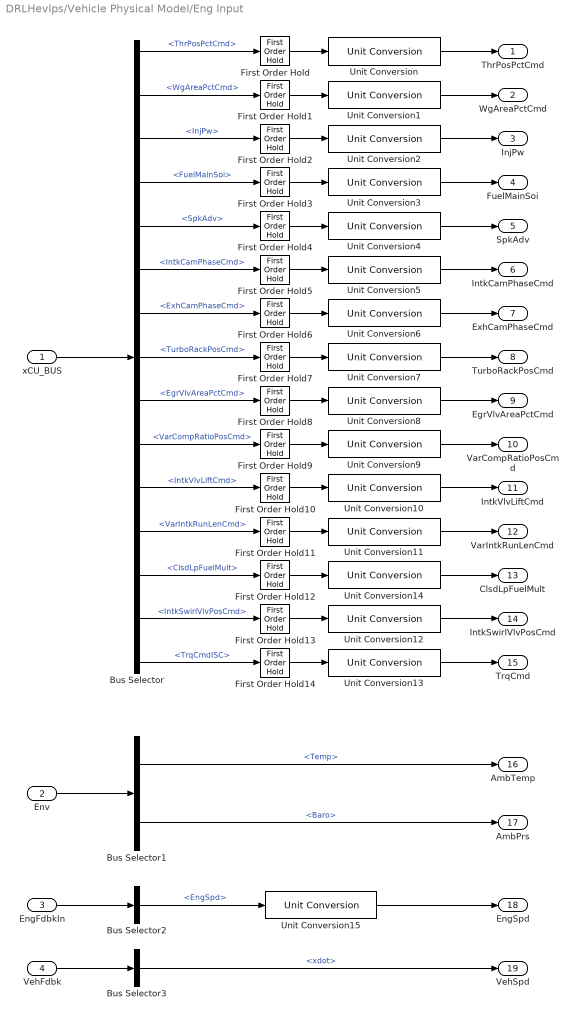
== system DRLHevIps/Vehicle Physical Model/Eng Input ==
  xCU_BUS : Inport
  Env : Inport  Port=2
  EngFdbkIn : Inport  Port=3
  VehFdbk : Inport  Port=4
  Bus Selector : BusSelector  OutputSignals=ECU_BUS.ThrPosPctCmd,ECU_BUS.WgAreaPctCmd,ECU_BUS.InjPw,ECU_BUS.FuelMainSoi,ECU_BUS.SpkAdv,ECU_BUS.IntkCamPhaseCmd,ECU_BUS.ExhCamPhaseCmd,ECU_BUS.TurboRackPosCmd,ECU_BUS.EgrVlvAreaPctCmd,ECU_BUS.VarCompRatioPosCmd,ECU_BUS.IntkVlvLiftCmd,ECU_BUS.VarIntkRunLenCmd,ECU_BUS.ClsdLpFuelMult,ECU_BUS.IntkSwirlVlvPosCmd,ECU_BUS.TrqCmdISC
  Bus Selector1 : BusSelector  OutputSignals=Temp,Baro
  Bus Selector2 : BusSelector  OutputSignals=EngSpd
  Bus Selector3 : BusSelector  OutputSignals=xdot
  First Order Hold{,1..14} (15 alike) : FirstOrderHold  ErrorTolerance=inf  AllowContinuousInput=on
  Unit Conversion{,1..15} (16 alike) : UnitConversion
  ThrPosPctCmd : Outport  VectorParamsAs1DForOutWhenUnconnected=off
  WgAreaPctCmd : Outport  Port=2  VectorParamsAs1DForOutWhenUnconnected=off
  InjPw : Outport  Port=3  VectorParamsAs1DForOutWhenUnconnected=off
  FuelMainSoi : Outport  Port=4  VectorParamsAs1DForOutWhenUnconnected=off
  SpkAdv : Outport  Port=5  VectorParamsAs1DForOutWhenUnconnected=off
  IntkCamPhaseCmd : Outport  Port=6  VectorParamsAs1DForOutWhenUnconnected=off
  ExhCamPhaseCmd : Outport  Port=7  VectorParamsAs1DForOutWhenUnconnected=off
  TurboRackPosCmd : Outport  Port=8  VectorParamsAs1DForOutWhenUnconnected=off
  EgrVlvAreaPctCmd : Outport  Port=9  VectorParamsAs1DForOutWhenUnconnected=off
  VarCompRatioPosCmd : Outport  Port=10  VectorParamsAs1DForOutWhenUnconnected=off
  IntkVlvLiftCmd : Outport  Port=11  VectorParamsAs1DForOutWhenUnconnected=off
  VarIntkRunLenCmd : Outport  Port=12  VectorParamsAs1DForOutWhenUnconnected=off
  ClsdLpFuelMult : Outport  Port=13  VectorParamsAs1DForOutWhenUnconnected=off
  IntkSwirlVlvPosCmd : Outport  Port=14  VectorParamsAs1DForOutWhenUnconnected=off
  TrqCmd : Outport  Port=15  VectorParamsAs1DForOutWhenUnconnected=off
  AmbTemp : Outport  Port=16  VectorParamsAs1DForOutWhenUnconnected=off
  AmbPrs : Outport  Port=17  VectorParamsAs1DForOutWhenUnconnected=off
  EngSpd : Outport  Port=18  VectorParamsAs1DForOutWhenUnconnected=off
  VehSpd : Outport  Port=19  VectorParamsAs1DForOutWhenUnconnected=off
  wires:
  Env/1 -> Bus Selector1/1
  Bus Selector1/2 -> AmbPrs/1  "<Baro>"
  EngFdbkIn/1 -> Bus Selector2/1
  Bus Selector2/1 -> Unit Conversion15/1  "<EngSpd>"
  Bus Selector1/1 -> AmbTemp/1  "<Temp>"
  VehFdbk/1 -> Bus Selector3/1
  Bus Selector3/1 -> VehSpd/1  "<xdot>"
  xCU_BUS/1 -> Bus Selector/1
  First Order Hold13/1 -> Unit Conversion12/1
  First Order Hold12/1 -> Unit Conversion14/1
  First Order Hold11/1 -> Unit Conversion11/1
  First Order Hold10/1 -> Unit Conversion10/1
  First Order Hold9/1 -> Unit Conversion9/1
  First Order Hold3/1 -> Unit Conversion3/1
  First Order Hold/1 -> Unit Conversion/1
  First Order Hold1/1 -> Unit Conversion1/1
  First Order Hold2/1 -> Unit Conversion2/1
  First Order Hold4/1 -> Unit Conversion4/1
  First Order Hold5/1 -> Unit Conversion5/1
  First Order Hold6/1 -> Unit Conversion6/1
  First Order Hold14/1 -> Unit Conversion13/1
  First Order Hold7/1 -> Unit Conversion7/1
  First Order Hold8/1 -> Unit Conversion8/1
  Bus Selector/1 -> First Order Hold/1  "<ThrPosPctCmd>"
  Bus Selector/2 -> First Order Hold1/1  "<WgAreaPctCmd>"
  Bus Selector/3 -> First Order Hold2/1  "<InjPw>"
  Bus Selector/4 -> First Order Hold3/1  "<FuelMainSoi>"
  Bus Selector/5 -> First Order Hold4/1  "<SpkAdv>"
  Bus Selector/6 -> First Order Hold5/1  "<IntkCamPhaseCmd>"
  Bus Selector/7 -> First Order Hold6/1  "<ExhCamPhaseCmd>"
  Bus Selector/8 -> First Order Hold7/1  "<TurboRackPosCmd>"
  Bus Selector/9 -> First Order Hold8/1  "<EgrVlvAreaPctCmd>"
  Bus Selector/10 -> First Order Hold9/1  "<VarCompRatioPosCmd>"
  Bus Selector/11 -> First Order Hold10/1  "<IntkVlvLiftCmd>"
  Bus Selector/12 -> First Order Hold11/1  "<VarIntkRunLenCmd>"
  Bus Selector/13 -> First Order Hold12/1  "<ClsdLpFuelMult>"
  Bus Selector/14 -> First Order Hold13/1  "<IntkSwirlVlvPosCmd>"
  Bus Selector/15 -> First Order Hold14/1  "<TrqCmdISC>"
  Unit Conversion11/1 -> VarIntkRunLenCmd/1
  Unit Conversion8/1 -> EgrVlvAreaPctCmd/1
  Unit Conversion12/1 -> IntkSwirlVlvPosCmd/1
  Unit Conversion14/1 -> ClsdLpFuelMult/1
  Unit Conversion/1 -> ThrPosPctCmd/1
  Unit Conversion1/1 -> WgAreaPctCmd/1
  Unit Conversion3/1 -> FuelMainSoi/1
  Unit Conversion2/1 -> InjPw/1
  Unit Conversion9/1 -> VarCompRatioPosCmd/1
  Unit Conversion4/1 -> SpkAdv/1
  Unit Conversion7/1 -> TurboRackPosCmd/1
  Unit Conversion13/1 -> TrqCmd/1
  Unit Conversion10/1 -> IntkVlvLiftCmd/1
  Unit Conversion6/1 -> ExhCamPhaseCmd/1
  Unit Conversion5/1 -> IntkCamPhaseCmd/1
  Unit Conversion15/1 -> EngSpd/1

== system DRLHevIps/Vehicle Physical Model/Eng Output ==
  EngTrq : Inport
  EngSpd : Inport  Port=2
  Map : Inport  Port=3
  Mat : Inport  Port=4
  ThrPosPct : Inport  Port=5
  WgAreaPct : Inport  Port=6
  IntkCamPhase : Inport  Port=7
  ExhCamPhase : Inport  Port=8
  TurboRackPos : Inport  Port=9
  EgrVlvAreaPct : Inport  Port=10
  VarCompRatioPos : Inport  Port=11
  IntkVlvLift : Inport  Port=12
  VarIntkRunLen : Inport  Port=13
  IntkSwirlVlvPos : Inport  Port=14
  FuelFlw : Inport  Port=15
  IntkPortFlow : Inport  Port=16
  NormAirChrg : Inport  Port=17
  ExhManGasTemp : Inport  Port=18
  Afr : Inport  Port=19
  TurboSpd : Inport  Port=20
  TurbPrsRatio : Inport  Port=21
  CompPrsRatio : Inport  Port=22
  TurbTempOut : Inport  Port=23
  CompTempOut : Inport  Port=24
  EgrPct : Inport  Port=25
  EgrMassFlwRate : Inport  Port=26
  EgrCoolerTempOut : Inport  Port=27
  IntercoolerTempOut : Inport  Port=28
  BSFC : Inport  Port=29
  TP HC : Inport  Port=30
  TP CO : Inport  Port=31
  TP NOx : Inport  Port=32
  TP CO2 : Inport  Port=33
  Iat : Inport  Port=34
  Ect : Inport  Port=35
  EgrVlvDeltaPrs : Inport  Port=36
  EgrVlvInTemp : Inport  Port=37
  Bus Creator1 : BusCreator  Inputs=37
  EngFdbkOut : Outport  VectorParamsAs1DForOutWhenUnconnected=off
  wires:
  VarIntkRunLen/1 -> Bus Creator1/13  "VarIntkRunLen"
  IntkVlvLift/1 -> Bus Creator1/12  "IntkVlvLift"
  VarCompRatioPos/1 -> Bus Creator1/11  "VarCompRatioPos"
  WgAreaPct/1 -> Bus Creator1/6  "WgAreaPct"
  TurboRackPos/1 -> Bus Creator1/9  "TurboRackPos"
  ThrPosPct/1 -> Bus Creator1/5  "ThrPosPct"
  EngTrq/1 -> Bus Creator1/1  "EngTrq"
  Mat/1 -> Bus Creator1/4  "Mat"
  Map/1 -> Bus Creator1/3  "Map"
  EngSpd/1 -> Bus Creator1/2  "EngSpd"
  Bus Creator1/1 -> EngFdbkOut/1  "EngFdbkOut"
  IntkCamPhase/1 -> Bus Creator1/7  "IntkCamPhase"
  ExhCamPhase/1 -> Bus Creator1/8  "ExhCamPhase"
  EgrVlvAreaPct/1 -> Bus Creator1/10  "EgrVlvAreaPct"
  IntkSwirlVlvPos/1 -> Bus Creator1/14  "IntkSwirlVlvPos"
  FuelFlw/1 -> Bus Creator1/15  "FuelFlw"
  IntkPortFlow/1 -> Bus Creator1/16  "IntkPortFlow"
  NormAirChrg/1 -> Bus Creator1/17  "NormAirChrg"
  ExhManGasTemp/1 -> Bus Creator1/18  "ExhManGasTemp"
  Afr/1 -> Bus Creator1/19  "Afr"
  TurboSpd/1 -> Bus Creator1/20  "TurboSpd"
  TurbPrsRatio/1 -> Bus Creator1/21  "TurbPrsRatio"
  CompPrsRatio/1 -> Bus Creator1/22  "CompPrsRatio"
  TurbTempOut/1 -> Bus Creator1/23  "TurbTempOut"
  CompTempOut/1 -> Bus Creator1/24  "CompTempOut"
  EgrPct/1 -> Bus Creator1/25  "EgrPct"
  EgrMassFlwRate/1 -> Bus Creator1/26  "EgrMassFlwRate"
  EgrCoolerTempOut/1 -> Bus Creator1/27  "EgrCoolerTempOut"
  IntercoolerTempOut/1 -> Bus Creator1/28  "IntercoolerTempOut"
  BSFC/1 -> Bus Creator1/29  "BSFC"
  TP HC/1 -> Bus Creator1/30  "TP HC"
  TP CO/1 -> Bus Creator1/31  "TP CO"
  TP NOx/1 -> Bus Creator1/32  "TP NOx"
  TP CO2/1 -> Bus Creator1/33  "TP CO2"
  Iat/1 -> Bus Creator1/34  "Iat"
  Ect/1 -> Bus Creator1/35  "Ect"
  EgrVlvDeltaPrs/1 -> Bus Creator1/36  "EgrVlvDeltaPrs"
  EgrVlvInTemp/1 -> Bus Creator1/37  "EgrVlvInTemp"

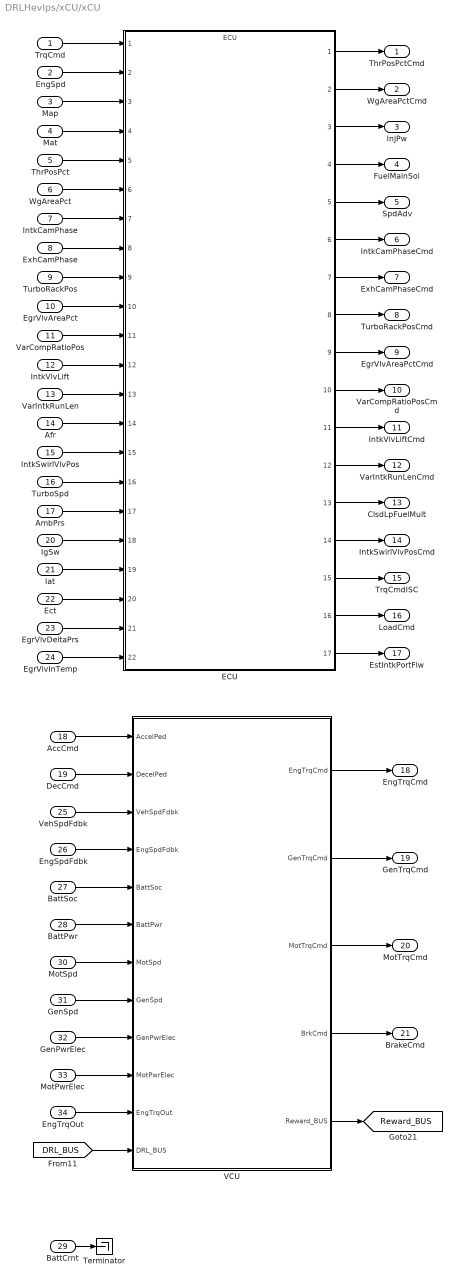
== system DRLHevIps/xCU/xCU ==
  TrqCmd : Inport
  EngSpd : Inport  Port=2
  Map : Inport  Port=3
  Mat : Inport  Port=4
  ThrPosPct : Inport  Port=5
  WgAreaPct : Inport  Port=6
  IntkCamPhase : Inport  Port=7
  ExhCamPhase : Inport  Port=8
  TurboRackPos : Inport  Port=9
  EgrVlvAreaPct : Inport  Port=10
  VarCompRatioPos : Inport  Port=11
  IntkVlvLift : Inport  Port=12
  VarIntkRunLen : Inport  Port=13
  Afr : Inport  Port=14
  IntkSwirlVlvPos : Inport  Port=15
  TurboSpd : Inport  Port=16
  AmbPrs : Inport  Port=17
  AccCmd : Inport  Port=18
  DecCmd : Inport  Port=19
  IgSw : Inport  Port=20
  Iat : Inport  Port=21
  Ect : Inport  Port=22
  EgrVlvDeltaPrs : Inport  Port=23
  EgrVlvInTemp : Inport  Port=24
  VehSpdFdbk : Inport  Port=25
  EngSpdFdbk : Inport  Port=26
  BattSoc : Inport  Port=27
  BattPwr : Inport  Port=28
  BattCrnt : Inport  Port=29
  MotSpd : Inport  Port=30
  GenSpd : Inport  Port=31
  GenPwrElec : Inport  Port=32
  MotPwrElec : Inport  Port=33
  EngTrqOut : Inport  Port=34
  ECU : ModelReference  ModelNameDialog=ECU.slx  ModelReferenceVersion=13.9
  Terminator : Terminator
  VCU : Subsystem  Variant=on  VariantActivationTime=inherit from Simulink.VariantControl
  ThrPosPctCmd : Outport  VectorParamsAs1DForOutWhenUnconnected=off
  WgAreaPctCmd : Outport  Port=2  VectorParamsAs1DForOutWhenUnconnected=off
  InjPw : Outport  Port=3  VectorParamsAs1DForOutWhenUnconnected=off
  FuelMainSoi : Outport  Port=4  VectorParamsAs1DForOutWhenUnconnected=off
  SpdAdv : Outport  Port=5  VectorParamsAs1DForOutWhenUnconnected=off
  IntkCamPhaseCmd : Outport  Port=6  VectorParamsAs1DForOutWhenUnconnected=off
  ExhCamPhaseCmd : Outport  Port=7  VectorParamsAs1DForOutWhenUnconnected=off
  TurboRackPosCmd : Outport  Port=8  VectorParamsAs1DForOutWhenUnconnected=off
  EgrVlvAreaPctCmd : Outport  Port=9  VectorParamsAs1DForOutWhenUnconnected=off
  VarCompRatioPosCmd : Outport  Port=10  VectorParamsAs1DForOutWhenUnconnected=off
  IntkVlvLiftCmd : Outport  Port=11  VectorParamsAs1DForOutWhenUnconnected=off
  VarIntkRunLenCmd : Outport  Port=12  VectorParamsAs1DForOutWhenUnconnected=off
  ClsdLpFuelMult : Outport  Port=13  VectorParamsAs1DForOutWhenUnconnected=off
  IntkSwirlVlvPosCmd : Outport  Port=14  VectorParamsAs1DForOutWhenUnconnected=off
  TrqCmdISC : Outport  Port=15  VectorParamsAs1DForOutWhenUnconnected=off
  LoadCmd : Outport  Port=16  VectorParamsAs1DForOutWhenUnconnected=off
  EstIntkPortFlw : Outport  Port=17  VectorParamsAs1DForOutWhenUnconnected=off
  EngTrqCmd : Outport  Port=18  VectorParamsAs1DForOutWhenUnconnected=off
  GenTrqCmd : Outport  Port=19  VectorParamsAs1DForOutWhenUnconnected=off
  MotTrqCmd : Outport  Port=20  VectorParamsAs1DForOutWhenUnconnected=off
  BrakeCmd : Outport  Port=21  VectorParamsAs1DForOutWhenUnconnected=off
  tag scope: Reward_BUS=global
  wires:
  VarCompRatioPos/1 -> ECU/11
  IntkVlvLift/1 -> ECU/12
  VarIntkRunLen/1 -> ECU/13
  Afr/1 -> ECU/14
  IntkSwirlVlvPos/1 -> ECU/15
  WgAreaPct/1 -> ECU/6
  ThrPosPct/1 -> ECU/5
  EgrVlvAreaPct/1 -> ECU/10
  TurboRackPos/1 -> ECU/9
  Mat/1 -> ECU/4
  Map/1 -> ECU/3
  EngSpd/1 -> ECU/2
  TrqCmd/1 -> ECU/1
  AmbPrs/1 -> ECU/17
  TurboSpd/1 -> ECU/16
  ExhCamPhase/1 -> ECU/8
  IntkCamPhase/1 -> ECU/7
  IgSw/1 -> ECU/18
  VCU/1(EngTrqCmd) -> EngTrqCmd/1
  VCU/3(MotTrqCmd) -> MotTrqCmd/1
  VCU/2(GenTrqCmd) -> GenTrqCmd/1
  VCU/4(BrkCmd) -> BrakeCmd/1
  VehSpdFdbk/1 -> VCU/3(VehSpdFdbk)
  AccCmd/1 -> VCU/1(AccelPed)
  DecCmd/1 -> VCU/2(DecelPed)
  EngSpdFdbk/1 -> VCU/4(EngSpdFdbk)
  BattPwr/1 -> VCU/6(BattPwr)
  BattSoc/1 -> VCU/5(BattSoc)
  MotSpd/1 -> VCU/7(MotSpd)
  BattCrnt/1 -> Terminator/1
  GenSpd/1 -> VCU/8(GenSpd)
  GenPwrElec/1 -> VCU/9(GenPwrElec)
  MotPwrElec/1 -> VCU/10(MotPwrElec)
  EngTrqOut/1 -> VCU/11(EngTrqOut)
  ECU/1 -> ThrPosPctCmd/1
  ECU/2 -> WgAreaPctCmd/1
  ECU/3 -> InjPw/1
  ECU/4 -> FuelMainSoi/1
  ECU/5 -> SpdAdv/1
  ECU/6 -> IntkCamPhaseCmd/1
  ECU/7 -> ExhCamPhaseCmd/1
  ECU/8 -> TurboRackPosCmd/1
  ECU/9 -> EgrVlvAreaPctCmd/1
  ECU/10 -> VarCompRatioPosCmd/1
  ECU/11 -> IntkVlvLiftCmd/1
  ECU/12 -> VarIntkRunLenCmd/1
  ECU/13 -> ClsdLpFuelMult/1
  ECU/14 -> IntkSwirlVlvPosCmd/1
  ECU/15 -> TrqCmdISC/1
  ECU/16 -> LoadCmd/1
  ECU/17 -> EstIntkPortFlw/1
  Iat/1 -> ECU/19
  Ect/1 -> ECU/20
  EgrVlvDeltaPrs/1 -> ECU/21
  EgrVlvInTemp/1 -> ECU/22
  [DRL_BUS] -> VCU/12(DRL_BUS)
  VCU/5(Reward_BUS) -> [Reward_BUS]
